simulink model "mj_IP_kalman"  (R2025b)
settings: Solver=VariableStepAuto  StartTime=0.0  StopTime=5  RelTol=1e-3
PostLoadFcn:
  | mj_IP_init
InitFcn:
  | mj_IP_init
values from neighbouring files (symbols this model uses):
  C = [1, 0, 0, 0]    [IP2_init.m]    (also in IP3_init.m; IP4_init.m; IP_init.m; mj_IP_init.m)
  D = 0    [IP2_init.m]    (also in IP3_init.m; IP4_init.m; IP_init.m; mj_IP_init.m)
  K = place(A, B, p)    [IP2_init.m]    (also in IP3_init.m; IP4_init.m; IP_init.m; mj_IP_init.m)
  kf = -1 / (C*((A - B*K) \ B))    [IP2_init.m]    (also in IP3_init.m; IP4_init.m; IP_init.m; mj_IP_init.m)
  sys_d = c2d(ss(A,B,C,D), 0.002, 'zoh')    [mj_IP_init.m]
undefined symbols (not defined in the file or in its folder): Discrete, Time
libraries: simulink x2, ctrlSharedLib x1, mjLib x1
settings Model: Creator=vmano  LastModifiedBy=Junch
settings OptimizationCC: ReuseModelBlockBuffer=off
settings ModelReferenceCC: EnableRefExpFcnMdlSchedulingChecks=on
settings SFSimCC: SimTargetLang=C++  SimDLTargetLibrary=mkl-dnn
settings RTWCC: GPUComputeCapability=3.5

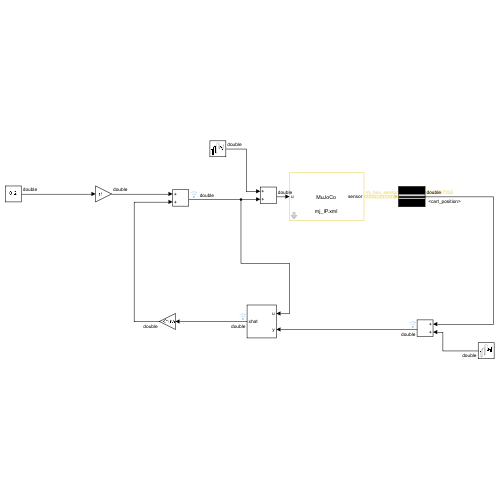
[thumbnail: Simulink's stored preview of the top-level diagram]
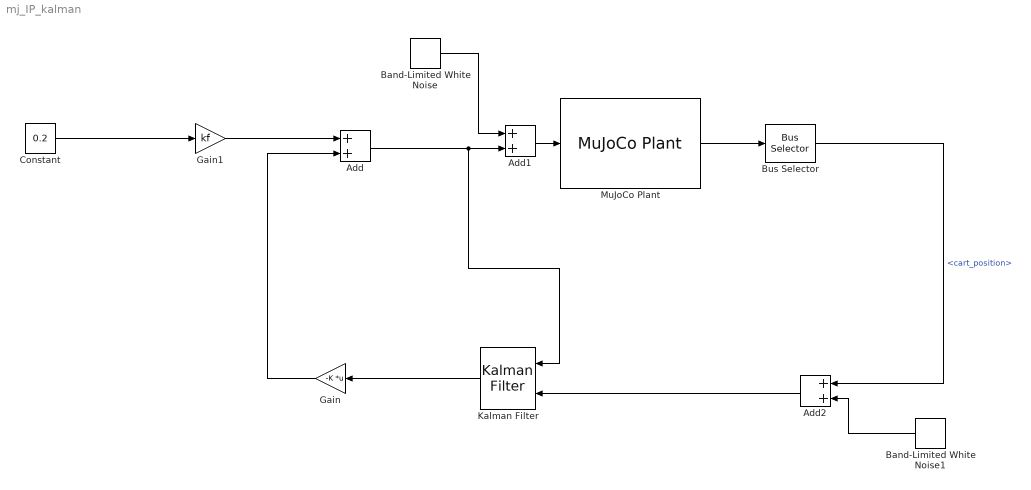
== system mj_IP_kalman ==
  Add : Sum
  Add1 : Sum
  Add2 : Sum
  Band-Limited White Noise : simulink/Sources/Band-Limited White Noise  Cov=[0.002]*0.2  Ts=0.002  seed=[23341]
  Band-Limited White Noise1 : simulink/Sources/Band-Limited White Noise  Cov=[0.002]*5e-6  Ts=0.002  seed=[23342]
  Bus Selector : BusSelector  OutputSignals=cart_position
  Constant : Constant  Value=0.2
  Gain : Gain  Gain=-K  Multiplication=Matrix(K*u) (u vector)
  Gain1 : Gain  Gain=kf
  Kalman Filter : ctrlSharedLib/Kalman Filter  TimeDomain=Discrete-Time  UseCurrentEstimator=on  ModelSource=Individual A, B, C, D matrices  ModelSourceVariable=ss(0.95,1,1,0,1)  A=sys_d.A  B=sys_d.B  C=C  D=D  NumberOfStates=1  NumberOfInputs=1  NumberOfOutputs=1  InitialEstimateSource=Dialog  X0=0  P0=10  UseK=off  UseGH=on  NumberOfProcessNoiseInputs=1  G=sys_d.B  TimeInvariantG=on  H=0  TimeInvariantH=on  Q=0.2  TimeInvariantQ=on  R=5e-6  TimeInvariantR=on  N=0  TimeInvariantN=on  AddInputPort=on  AddEnablePort=off  OutputEstimatedY=off  OutputP=off  Ts=-1
  MuJoCo Plant : mjLib/MuJoCo Plant  controlBus=[]  sensorBus=mj_bus_sensor_7979902499018342666  controlLength=[]  sensorLength=[]  rgbLength=[]  depthLength=[]  sampleTime=0.002  xmlFileRel=mj_IP.xml  xmlFile=E:\robotics\simulink\mj_IP.xml  renderingType=Global  vsync=off  visualFPS=60  zoomLevel=1  windowWidth=1200  windowHeight=800  showSiteTrajectory=off  znear=0.023333  zfar=116.6667  cameraOutputEnabled=off  cameraSampleTime=0.050  rgbOutOption=on  depthOutOption=off  controlInterfaceType=Vector
      settings: SourceProductName=MuJoCo Simulator
  wires:
  MuJoCo Plant/1 -> Bus Selector/1
  Bus Selector/1 -> Add2/1  "<cart_position>"
  Gain/1 -> Add/2
  Kalman Filter/1 -> Gain/1
  Gain1/1 -> Add/1
  Add/1 -> Kalman Filter/1, Add1/2
  Constant/1 -> Gain1/1
  Add1/1 -> MuJoCo Plant/1
  Band-Limited White Noise/1 -> Add1/1
  Band-Limited White Noise1/1 -> Add2/2
  Add2/1 -> Kalman Filter/2
